simulink model "PI_Capacitors"  (R2023a)
settings: Solver=VariableStepAuto  StartTime=0.0  StopTime=10.0  RelTol=1e-3
libraries: fl_lib x38, nesl_utility x12
settings Model: Creator=Shahd Bassem  LastModifiedBy=Shahd Bassem

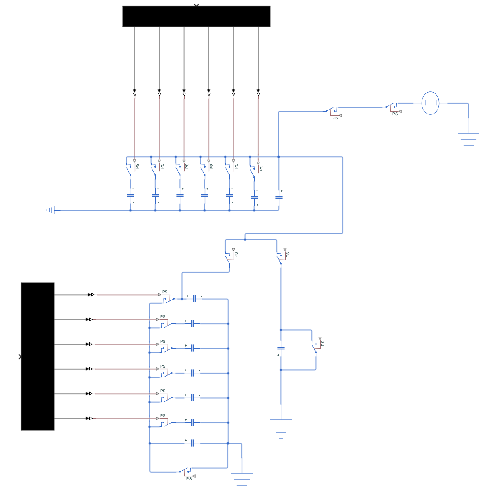
[thumbnail: Simulink's stored preview of the top-level diagram]
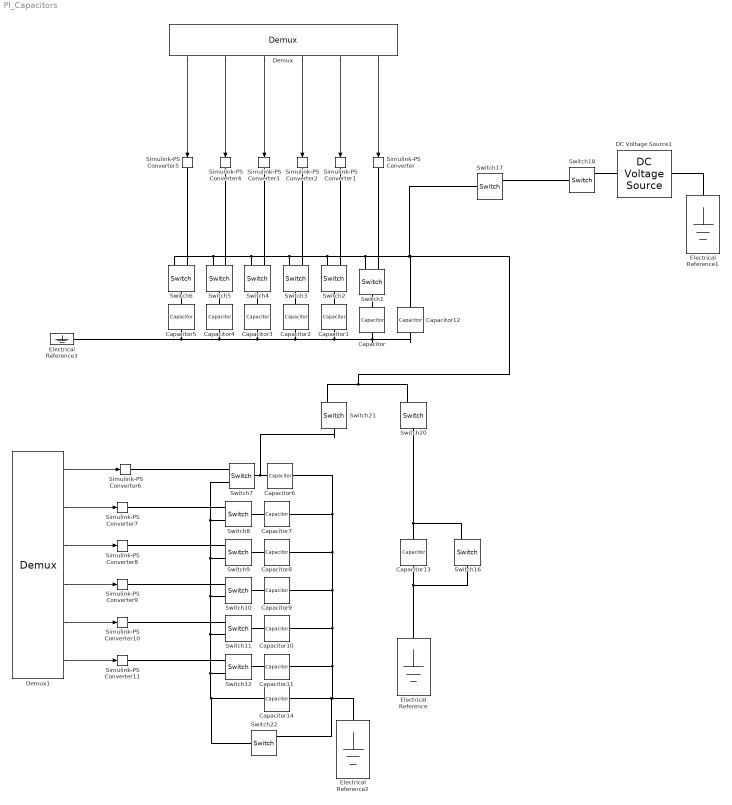
== system PI_Capacitors ==
  Capacitor : fl_lib/Electrical/Electrical Elements/Capacitor  c=32e-15 F  r=1e-6 Ohm  g=0 1/Ohm  i_specify=off  i_priority=None  i=0 A  i_nominal_specify=off  i_nominal_unit=A  i_nominal_value=1  v_specify=off  v_priority=None  v=0 V  v_nominal_specify=off  v_nominal_unit=V  v_nominal_value=1  vc_specify=off  vc_priority=High  vc=0 V  vc_nominal_specify=off  vc_nominal_unit=V  vc_nominal_value=1
  Capacitor1 : fl_lib/Electrical/Electrical Elements/Capacitor  c=16e-15 F  r=1e-6 Ohm  g=0 1/Ohm  i_specify=off  i_priority=None  i=0 A  i_nominal_specify=off  i_nominal_unit=A  i_nominal_value=1  v_specify=off  v_priority=None  v=0 V  v_nominal_specify=off  v_nominal_unit=V  v_nominal_value=1  vc_specify=off  vc_priority=High  vc=0 V  vc_nominal_specify=off  vc_nominal_unit=V  vc_nominal_value=1
  Capacitor10 : fl_lib/Electrical/Electrical Elements/Capacitor  c=16e-15 F  r=1e-6 Ohm  g=0 1/Ohm  i_specify=off  i_priority=None  i=0 A  i_nominal_specify=off  i_nominal_unit=A  i_nominal_value=1  v_specify=off  v_priority=None  v=0 V  v_nominal_specify=off  v_nominal_unit=V  v_nominal_value=1  vc_specify=off  vc_priority=High  vc=0 V  vc_nominal_specify=off  vc_nominal_unit=V  vc_nominal_value=1
  Capacitor11 : fl_lib/Electrical/Electrical Elements/Capacitor  c=32e-15 F  r=1e-6 Ohm  g=0 1/Ohm  i_specify=off  i_priority=None  i=0 A  i_nominal_specify=off  i_nominal_unit=A  i_nominal_value=1  v_specify=off  v_priority=None  v=0 V  v_nominal_specify=off  v_nominal_unit=V  v_nominal_value=1  vc_specify=off  vc_priority=High  vc=0 V  vc_nominal_specify=off  vc_nominal_unit=V  vc_nominal_value=1
  Capacitor12 : fl_lib/Electrical/Electrical Elements/Capacitor  c=37e-15 F  r=1e-6 Ohm  g=0 1/Ohm  i_specify=off  i_priority=None  i=0 A  i_nominal_specify=off  i_nominal_unit=A  i_nominal_value=1  v_specify=off  v_priority=None  v=0 V  v_nominal_specify=off  v_nominal_unit=V  v_nominal_value=1  vc_specify=off  vc_priority=High  vc=0 V  vc_nominal_specify=off  vc_nominal_unit=V  vc_nominal_value=1
  Capacitor13 : fl_lib/Electrical/Electrical Elements/Capacitor  c=20e-15 F  r=1e-6 Ohm  g=0 1/Ohm  i_specify=off  i_priority=None  i=0 A  i_nominal_specify=off  i_nominal_unit=A  i_nominal_value=1  v_specify=off  v_priority=None  v=0 V  v_nominal_specify=off  v_nominal_unit=V  v_nominal_value=1  vc_specify=off  vc_priority=High  vc=0 V  vc_nominal_specify=off  vc_nominal_unit=V  vc_nominal_value=1
  Capacitor14 : fl_lib/Electrical/Electrical Elements/Capacitor  c=10e-15 F  r=1e-6 Ohm  g=0 1/Ohm  i_specify=off  i_priority=None  i=0 A  i_nominal_specify=off  i_nominal_unit=A  i_nominal_value=1  v_specify=off  v_priority=None  v=0 V  v_nominal_specify=off  v_nominal_unit=V  v_nominal_value=1  vc_specify=off  vc_priority=High  vc=0 V  vc_nominal_specify=off  vc_nominal_unit=V  vc_nominal_value=1
  Capacitor2 : fl_lib/Electrical/Electrical Elements/Capacitor  c=8e-15 F  r=1e-6 Ohm  g=0 1/Ohm  i_specify=off  i_priority=None  i=0 A  i_nominal_specify=off  i_nominal_unit=A  i_nominal_value=1  v_specify=off  v_priority=None  v=0 V  v_nominal_specify=off  v_nominal_unit=V  v_nominal_value=1  vc_specify=off  vc_priority=High  vc=0 V  vc_nominal_specify=off  vc_nominal_unit=V  vc_nominal_value=1
  Capacitor3 : fl_lib/Electrical/Electrical Elements/Capacitor  c=4e-15 F  r=1e-6 Ohm  g=0 1/Ohm  i_specify=off  i_priority=None  i=0 A  i_nominal_specify=off  i_nominal_unit=A  i_nominal_value=1  v_specify=off  v_priority=None  v=0 V  v_nominal_specify=off  v_nominal_unit=V  v_nominal_value=1  vc_specify=off  vc_priority=High  vc=0 V  vc_nominal_specify=off  vc_nominal_unit=V  vc_nominal_value=1
  Capacitor4 : fl_lib/Electrical/Electrical Elements/Capacitor  c=2e-15 F  r=1e-6 Ohm  g=0 1/Ohm  i_specify=off  i_priority=None  i=0 A  i_nominal_specify=off  i_nominal_unit=A  i_nominal_value=1  v_specify=off  v_priority=None  v=0 V  v_nominal_specify=off  v_nominal_unit=V  v_nominal_value=1  vc_specify=off  vc_priority=High  vc=0 V  vc_nominal_specify=off  vc_nominal_unit=V  vc_nominal_value=1
  Capacitor5 : fl_lib/Electrical/Electrical Elements/Capacitor  c=1e-15 F  r=1e-6 Ohm  g=0 1/Ohm  i_specify=off  i_priority=None  i=0 A  i_nominal_specify=off  i_nominal_unit=A  i_nominal_value=1  v_specify=off  v_priority=None  v=0 V  v_nominal_specify=off  v_nominal_unit=V  v_nominal_value=1  vc_specify=off  vc_priority=High  vc=0 V  vc_nominal_specify=off  vc_nominal_unit=V  vc_nominal_value=1
  Capacitor6 : fl_lib/Electrical/Electrical Elements/Capacitor  c=1e-15 F  r=1e-6 Ohm  g=0 1/Ohm  i_specify=off  i_priority=None  i=0 A  i_nominal_specify=off  i_nominal_unit=A  i_nominal_value=1  v_specify=off  v_priority=None  v=0 V  v_nominal_specify=off  v_nominal_unit=V  v_nominal_value=1  vc_specify=off  vc_priority=High  vc=0 V  vc_nominal_specify=off  vc_nominal_unit=V  vc_nominal_value=1
  Capacitor7 : fl_lib/Electrical/Electrical Elements/Capacitor  c=2e-15 F  r=1e-6 Ohm  g=0 1/Ohm  i_specify=off  i_priority=None  i=0 A  i_nominal_specify=off  i_nominal_unit=A  i_nominal_value=1  v_specify=off  v_priority=None  v=0 V  v_nominal_specify=off  v_nominal_unit=V  v_nominal_value=1  vc_specify=off  vc_priority=High  vc=0 V  vc_nominal_specify=off  vc_nominal_unit=V  vc_nominal_value=1
  Capacitor8 : fl_lib/Electrical/Electrical Elements/Capacitor  c=4e-15 F  r=1e-6 Ohm  g=0 1/Ohm  i_specify=off  i_priority=None  i=0 A  i_nominal_specify=off  i_nominal_unit=A  i_nominal_value=1  v_specify=off  v_priority=None  v=0 V  v_nominal_specify=off  v_nominal_unit=V  v_nominal_value=1  vc_specify=off  vc_priority=High  vc=0 V  vc_nominal_specify=off  vc_nominal_unit=V  vc_nominal_value=1
  Capacitor9 : fl_lib/Electrical/Electrical Elements/Capacitor  c=8e-15 F  r=1e-6 Ohm  g=0 1/Ohm  i_specify=off  i_priority=None  i=0 A  i_nominal_specify=off  i_nominal_unit=A  i_nominal_value=1  v_specify=off  v_priority=None  v=0 V  v_nominal_specify=off  v_nominal_unit=V  v_nominal_value=1  vc_specify=off  vc_priority=High  vc=0 V  vc_nominal_specify=off  vc_nominal_unit=V  vc_nominal_value=1
  DC Voltage Source1 : fl_lib/Electrical/Electrical Sources/DC Voltage Source  v0=1 V
  Demux : Demux  Outputs=6
  Demux1 : Demux  Outputs=6
  Electrical Reference{,1..3} (4 alike) : fl_lib/Electrical/Electrical Elements/Electrical Reference
  Simulink-PS Converter{,1..11} (12 alike) : nesl_utility/Simulink-PS Converter  PhysicalDomain=network_engine_domain  SubClassName=ps_input  LeftPortType=input  RightPortType=output  PseudoPeriodic=off  Frequencies=[]  NoiseDistribution=none  NoiseParameters=[]  Unit=1  AffineConversion=off  FilteringAndDerivatives=provide  SimscapeFilterOrder=1  InputFilterTimeConstant=0.001  UdotUserProvided=0
  Switch{1..12,16..18,20..22} (18 alike) : fl_lib/Electrical/Electrical Elements/Switch  R_closed=0.01 Ohm  G_open=1e-8 1/Ohm  Threshold=0.5  i_specify=off  i_priority=None  i=0 A  i_nominal_specify=off  i_nominal_unit=A  i_nominal_value=1  v_specify=off  v_priority=None  v=0 V  v_nominal_specify=off  v_nominal_unit=V  v_nominal_value=1
  wires:
  Demux1/2 -> Simulink-PS Converter7/1
  Demux1/3 -> Simulink-PS Converter8/1
  Demux1/1 -> Simulink-PS Converter6/1
  Demux1/6 -> Simulink-PS Converter11/1
  Demux1/5 -> Simulink-PS Converter10/1
  Demux1/4 -> Simulink-PS Converter9/1
  Demux/5 -> Simulink-PS Converter1/1
  Demux/4 -> Simulink-PS Converter2/1
  Demux/1 -> Simulink-PS Converter5/1
  Demux/2 -> Simulink-PS Converter4/1
  Demux/3 -> Simulink-PS Converter3/1
  Demux/6 -> Simulink-PS Converter/1
  connections:
  Switch1/LConn1 -- Capacitor/LConn1
  Simulink-PS Converter/RConn1 -- Switch1/RConn1
  Simulink-PS Converter1/RConn1 -- Switch2/RConn1
  Switch2/LConn1 -- Capacitor1/LConn1
  Simulink-PS Converter2/RConn1 -- Switch3/RConn1
  Switch3/LConn1 -- Capacitor2/LConn1
  Simulink-PS Converter3/RConn1 -- Switch4/RConn1
  Switch4/LConn1 -- Capacitor3/LConn1
  Simulink-PS Converter4/RConn1 -- Switch5/RConn1
  Switch5/LConn1 -- Capacitor4/LConn1
  Simulink-PS Converter5/RConn1 -- Switch6/RConn1
  Switch6/LConn1 -- Capacitor5/LConn1
  Switch7/RConn2 -- Switch11/RConn2 -- Switch22/LConn1 -- Capacitor14/LConn1 -- Switch12/RConn2 -- Switch10/RConn2 -- Switch9/RConn2 -- Switch8/RConn2
  Capacitor6/RConn1 -- Capacitor9/RConn1 -- Switch22/RConn2 -- Capacitor14/RConn1 -- Electrical Reference2/LConn1 -- Capacitor11/RConn1 -- Capacitor10/RConn1 -- Capacitor8/RConn1 -- Capacitor7/RConn1
  Simulink-PS Converter9/RConn1 -- Switch10/RConn1
  Simulink-PS Converter11/RConn1 -- Switch12/RConn1
  Switch8/LConn1 -- Capacitor7/LConn1
  Switch12/LConn1 -- Capacitor11/LConn1
  Switch10/LConn1 -- Capacitor9/LConn1
  Simulink-PS Converter6/RConn1 -- Switch7/RConn1
  Simulink-PS Converter10/RConn1 -- Switch11/RConn1
  Switch7/LConn1 -- Capacitor6/LConn1 -- Switch21/LConn1
  Simulink-PS Converter7/RConn1 -- Switch8/RConn1
  Switch9/LConn1 -- Capacitor8/LConn1
  Simulink-PS Converter8/RConn1 -- Switch9/RConn1
  Switch11/LConn1 -- Capacitor10/LConn1
  Electrical Reference/LConn1 -- Switch16/LConn1 -- Capacitor13/LConn1
  Switch17/RConn2 -- Switch18/LConn1
  Switch18/RConn2 -- DC Voltage Source1/LConn1
  DC Voltage Source1/RConn1 -- Electrical Reference1/LConn1
  Switch16/RConn2 -- Capacitor13/RConn1 -- Switch20/LConn1
  Capacitor/RConn1 -- Capacitor12/RConn1 -- Electrical Reference3/LConn1 -- Capacitor5/RConn1 -- Capacitor4/RConn1 -- Capacitor3/RConn1 -- Capacitor2/RConn1 -- Capacitor1/RConn1
  Switch6/RConn2 -- Switch20/RConn2 -- Switch21/RConn2 -- Capacitor12/LConn1 -- Switch17/LConn1 -- Switch1/RConn2 -- Switch2/RConn2 -- Switch3/RConn2 -- Switch4/RConn2 -- Switch5/RConn2
